simulink model "PlantVDBS1"  (R2023a)
settings: Solver=VariableStepAuto  StartTime=0.0  StopTime=10  MaxStep=0.002  RelTol=1e-6
undefined symbols (not defined in the file): c, C, C_alpha_f, C_col, C_r, E, e_c, F_zf, F_zr, J_col, K, l_f, l_r, m, n_st, t_0, T_f
libraries: autolibshared x1
settings Model: Creator=Tan_Tram  LastModifiedBy=Tan_Tram

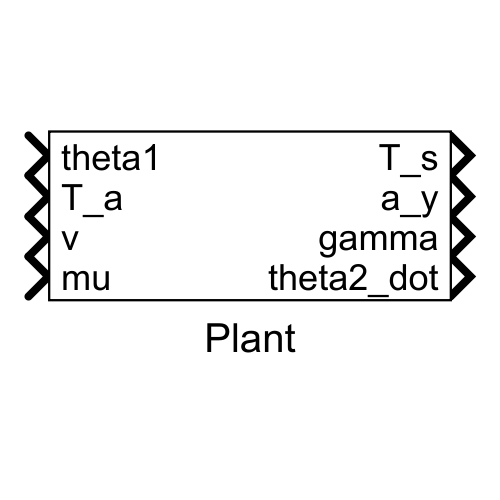
[thumbnail: Simulink's stored preview of the top-level diagram]
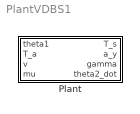
== system PlantVDBS1 ==
  Plant : Subsystem

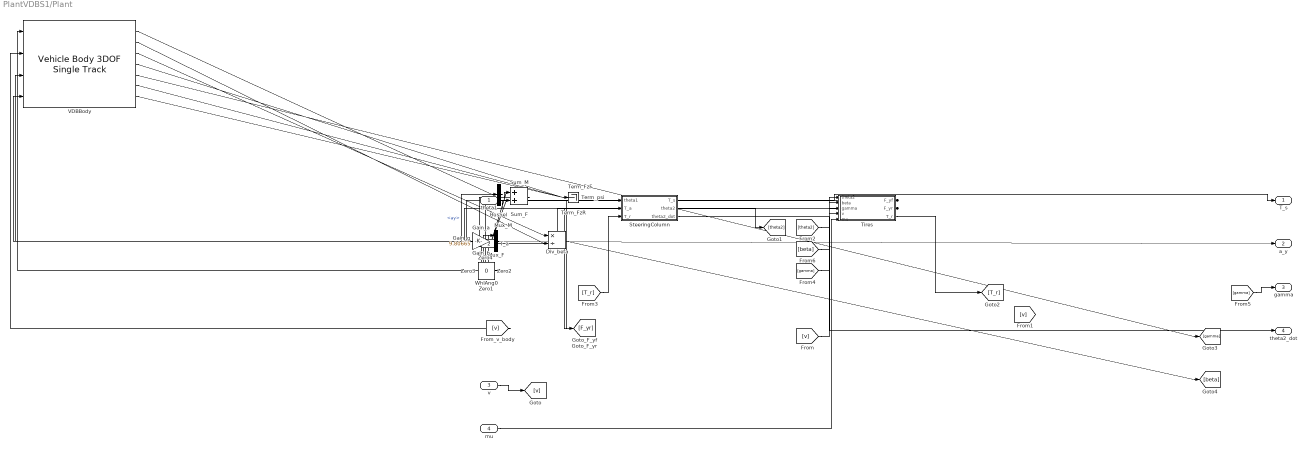
== system PlantVDBS1/Plant ==
  theta1 : Inport
  T_a : Inport  Port=2
  v : Inport  Port=3
  mu : Inport  Port=4
  BusSel : BusSelector  OutputSignals=BdyFrm.Cg.Acc.ay
  Div_beta : Product  Inputs=*/
  Gain_a : Gain  Gain=l_f
  Gain_b : Gain  Gain=l_r
  Gain_g : Gain  Gain=9.80665
  Mux_F : Mux  Inputs=3
  Mux_M : Mux  Inputs=3
  SteeringColumn : Subsystem
  Sum_F : Sum
  Sum_M : Sum  Inputs=+-
  Term_FzF : Terminator
  Term_FzR : Terminator
  Term_psi : Terminator
  Tires : Subsystem
  VDBBody : autolibshared/Vehicle Body 3DOF Single Track  trackMode=Single (bicycle)  inputMode=External longitudinal velocity  frontSteerMode=on  rearSteerMode=off  windMode=off  muMode=off  extFMode=on  extMMode=on  htchFMode=off  htchMMode=off  extXo=off  extpsio=off  extxdoto=off  extro=off  extYo=off  extTamb=off  extydoto=off  aMode=2  NF=2  NR=2  m=m  a=l_f  b=l_r  h=0.35  dh=1  hh=0.2  X_o=0  xdot_o=vdb_v0  CalphaMode=off  sigmaMode=off  d=0  hl=0  w=[1.4,1.4]  Cy_f=0  Cy_r=0  sigma_f=.1  sigma_r=.1  alpha_f_brk=[-.1 .1]  Cy_f_data=[-9e3 9e3]  alpha_r_brk=[-.1 .1]  Cy_r_data=[-9e3 9e3]  Y_o=0  ydot_o=0  Izz=Iz  psi_o=0  r_o=0  Af=2  Cd=0  Cl=0  Cpm=0  beta_w=[0 0.01:0.01:0.3]  Cs=[0 0 0 0 0 0 0 0 0 0 0 0 0 0 0 0 0 0 0 0 0 0 0 0 0 0 0 0 0 0 0]  Cym=[0 0 0 0 0 0 0 0 0 0 0 0 0 0 0 0 0 0 0 0 0 0 0 0 0 0 0 0 0 0 0]  Pabs=101325  Tair=273  g=9.81  mu=1  xdot_tol=.01  Fznom=5000  Fxtire_sat=7e4  Fytire_sat=7e4  longOff=0  latOff=0  vertOff=0  wrapAng=off
  WhlAng0 : Constant  Value=0
  Zero{1..4} (4 alike) : Constant  Value=0
  T_s : Outport
  a_y : Outport  Port=2
  gamma : Outport  Port=3
  theta2_dot : Outport  Port=4
  wires:
  [beta] -> Tires/2(beta)
  [gamma] -> gamma/1
  [gamma] -> Tires/3(gamma)
  [T_r] -> SteeringColumn/3(T_r)
  Tires/3(T_r) -> [T_r]
  [theta2] -> Tires/1(theta2)
  SteeringColumn/2(theta2) -> [theta2]
  [v] -> Tires/4(v)
  v/1 -> [v]
  SteeringColumn/3(theta2_dot) -> theta2_dot/1
  SteeringColumn/1(T_s) -> T_s/1
  mu/1 -> Tires/5(mu)
  T_a/1 -> SteeringColumn/2(T_a)
  theta1/1 -> SteeringColumn/1(theta1)
  Tires/1(F_yf) -> [F_yf], Sum_F/1, Gain_a/1
  Tires/2(F_yr) -> [F_yr], Sum_F/2, Gain_b/1
  Zero1/1 -> Mux_F/1
  Sum_F/1 -> Mux_F/2
  Zero2/1 -> Mux_F/3
  Gain_a/1 -> Sum_M/1
  Gain_b/1 -> Sum_M/2
  Zero3/1 -> Mux_M/1
  Zero4/1 -> Mux_M/2
  Sum_M/1 -> Mux_M/3
  WhlAng0/1 -> VDBBody/1
  Mux_F/1 -> VDBBody/3
  Mux_M/1 -> VDBBody/4
  [v] -> VDBBody/2
  VDBBody/3 -> Div_beta/1
  VDBBody/2 -> Div_beta/2
  Div_beta/1 -> [beta]
  VDBBody/5 -> [gamma]
  VDBBody/1 -> BusSel/1
  BusSel/1 -> Gain_g/1  "<ay>"
  Gain_g/1 -> a_y/1
  VDBBody/4 -> Term_psi/1
  VDBBody/6 -> Term_FzF/1
  VDBBody/7 -> Term_FzR/1

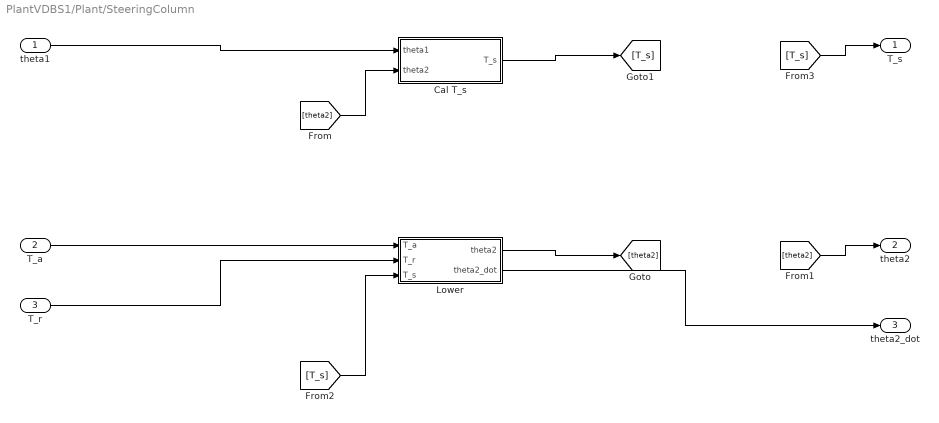
== system PlantVDBS1/Plant/SteeringColumn ==
  theta1 : Inport
  T_a : Inport  Port=2
  T_r : Inport  Port=3
  Cal T_s : Subsystem
  Lower : Subsystem
  T_s : Outport
  theta2 : Outport  Port=2
  theta2_dot : Outport  Port=3
  wires:
  theta1/1 -> Cal T_s/1(theta1)
  T_a/1 -> Lower/1(T_a)
  T_r/1 -> Lower/2(T_r)
  Lower/2(theta2_dot) -> theta2_dot/1
  Lower/1(theta2) -> [theta2]
  [theta2] -> Cal T_s/2(theta2)
  [theta2] -> theta2/1
  Cal T_s/1(T_s) -> [T_s]
  [T_s] -> Lower/3(T_s)
  [T_s] -> T_s/1

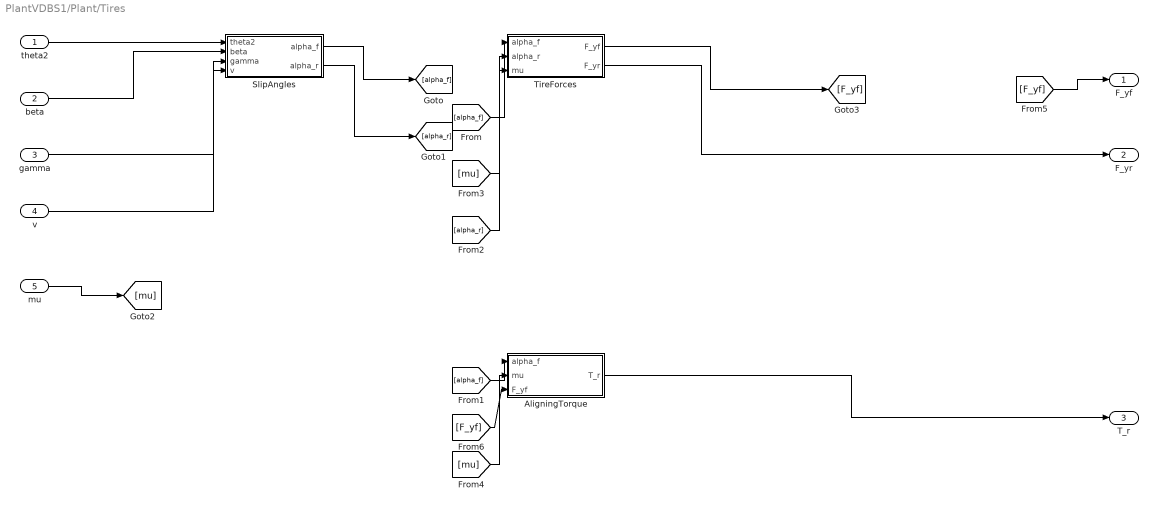
== system PlantVDBS1/Plant/Tires ==
  theta2 : Inport
  beta : Inport  Port=2
  gamma : Inport  Port=3
  v : Inport  Port=4
  mu : Inport  Port=5
  AligningTorque : Subsystem
  SlipAngles : Subsystem
  TireForces : Subsystem
  F_yf : Outport
  F_yr : Outport  Port=2
  T_r : Outport  Port=3
  wires:
  theta2/1 -> SlipAngles/1(theta2)
  beta/1 -> SlipAngles/2(beta)
  gamma/1 -> SlipAngles/3(gamma)
  v/1 -> SlipAngles/4(v)
  SlipAngles/1(alpha_f) -> [alpha_f]
  [alpha_f] -> TireForces/1(alpha_f)
  [alpha_f] -> AligningTorque/1(alpha_f)
  SlipAngles/2(alpha_r) -> [alpha_r]
  [alpha_r] -> TireForces/2(alpha_r)
  mu/1 -> [mu]
  [mu] -> TireForces/3(mu)
  [mu] -> AligningTorque/2(mu)
  TireForces/1(F_yf) -> [F_yf]
  [F_yf] -> F_yf/1
  [F_yf] -> AligningTorque/3(F_yf)
  TireForces/2(F_yr) -> F_yr/1
  AligningTorque/1(T_r) -> T_r/1

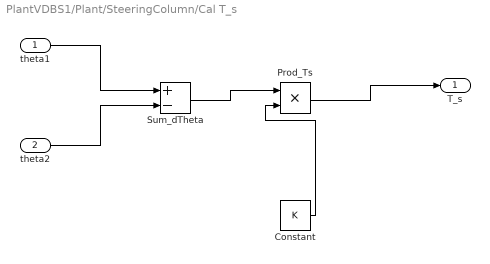
== system PlantVDBS1/Plant/SteeringColumn/Cal T_s ==
  theta1 : Inport
  theta2 : Inport  Port=2
  Constant : Constant  Value=K
  Prod_Ts : Product  Inputs=**
  Sum_dTheta : Sum  Inputs=+-
  T_s : Outport
  wires:
  theta1/1 -> Sum_dTheta/1
  theta2/1 -> Sum_dTheta/2
  Sum_dTheta/1 -> Prod_Ts/1
  Constant/1 -> Prod_Ts/2
  Prod_Ts/1 -> T_s/1

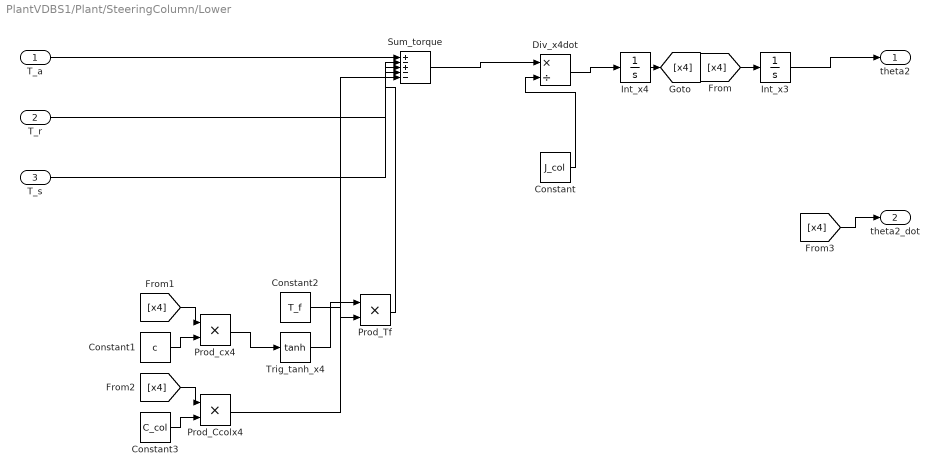
== system PlantVDBS1/Plant/SteeringColumn/Lower ==
  T_a : Inport
  T_r : Inport  Port=2
  T_s : Inport  Port=3
  Constant : Constant  Value=J_col
  Constant1 : Constant  Value=c
  Constant2 : Constant  Value=T_f
  Constant3 : Constant  Value=C_col
  Div_x4dot : Product  Inputs=*/
  Int_x3 : Integrator
  Int_x4 : Integrator
  Prod_Ccolx4 : Product  Inputs=**
  Prod_Tf : Product  Inputs=**
  Prod_cx4 : Product  Inputs=**
  Sum_torque : Sum  Inputs=+-+--
  Trig_tanh_x4 : Trigonometry  Operator=tanh
  theta2 : Outport
  theta2_dot : Outport  Port=2
  wires:
  Int_x4/1 -> [x4]
  [x4] -> Prod_cx4/1
  Constant1/1 -> Prod_cx4/2
  Prod_cx4/1 -> Trig_tanh_x4/1
  Trig_tanh_x4/1 -> Prod_Tf/1
  Constant2/1 -> Prod_Tf/2
  [x4] -> Prod_Ccolx4/1
  Constant3/1 -> Prod_Ccolx4/2
  T_a/1 -> Sum_torque/1
  T_r/1 -> Sum_torque/2
  T_s/1 -> Sum_torque/3
  Prod_Tf/1 -> Sum_torque/4
  Prod_Ccolx4/1 -> Sum_torque/5
  Sum_torque/1 -> Div_x4dot/1
  Constant/1 -> Div_x4dot/2
  Div_x4dot/1 -> Int_x4/1
  [x4] -> Int_x3/1
  Int_x3/1 -> theta2/1
  [x4] -> theta2_dot/1

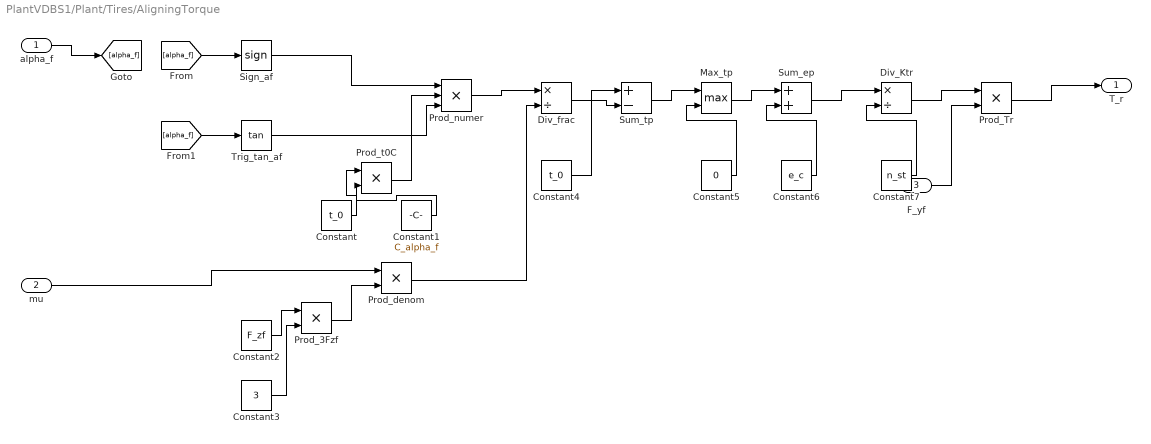
== system PlantVDBS1/Plant/Tires/AligningTorque ==
  alpha_f : Inport
  mu : Inport  Port=2
  F_yf : Inport  Port=3
  Constant : Constant  Value=t_0
  Constant1 : Constant  Value=C_alpha_f
  Constant2 : Constant  Value=F_zf
  Constant3 : Constant  Value=3
  Constant4 : Constant  Value=t_0
  Constant5 : Constant  Value=0
  Constant6 : Constant  Value=e_c
  Constant7 : Constant  Value=n_st
  Div_Ktr : Product  Inputs=*/
  Div_frac : Product  Inputs=*/
  Max_tp : MinMax  Function=max  Inputs=2
  Prod_3Fzf : Product  Inputs=**
  Prod_Tr : Product  Inputs=**
  Prod_denom : Product  Inputs=**
  Prod_numer : Product  Inputs=***
  Prod_t0C : Product  Inputs=**
  Sign_af : Signum
  Sum_ep : Sum
  Sum_tp : Sum  Inputs=+-
  Trig_tan_af : Trigonometry  Operator=tan
  T_r : Outport
  wires:
  alpha_f/1 -> [alpha_f]
  [alpha_f] -> Sign_af/1
  [alpha_f] -> Trig_tan_af/1
  Constant/1 -> Prod_t0C/1
  Constant1/1 -> Prod_t0C/2
  Sign_af/1 -> Prod_numer/1
  Prod_t0C/1 -> Prod_numer/2
  Trig_tan_af/1 -> Prod_numer/3
  Constant2/1 -> Prod_3Fzf/1
  Constant3/1 -> Prod_3Fzf/2
  mu/1 -> Prod_denom/1
  Prod_3Fzf/1 -> Prod_denom/2
  Prod_numer/1 -> Div_frac/1
  Prod_denom/1 -> Div_frac/2
  Constant4/1 -> Sum_tp/1
  Div_frac/1 -> Sum_tp/2
  Sum_tp/1 -> Max_tp/1
  Constant5/1 -> Max_tp/2
  Max_tp/1 -> Sum_ep/1
  Constant6/1 -> Sum_ep/2
  Sum_ep/1 -> Div_Ktr/1
  Constant7/1 -> Div_Ktr/2
  Div_Ktr/1 -> Prod_Tr/1
  F_yf/1 -> Prod_Tr/2
  Prod_Tr/1 -> T_r/1

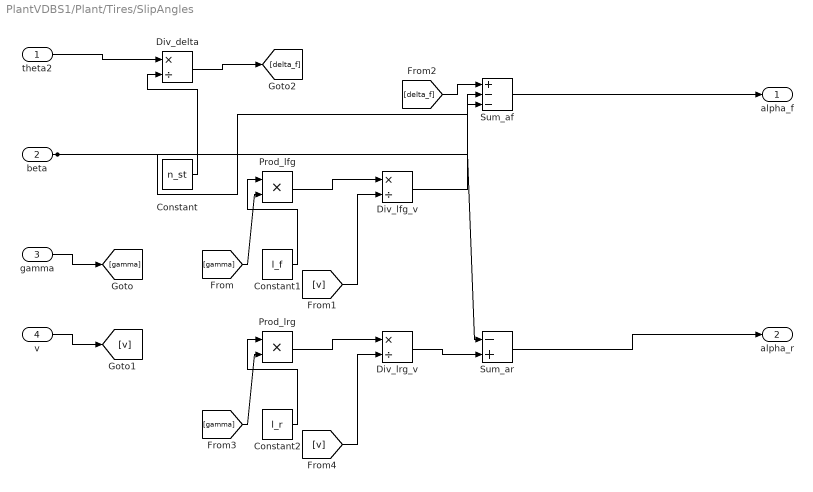
== system PlantVDBS1/Plant/Tires/SlipAngles ==
  theta2 : Inport
  beta : Inport  Port=2
  gamma : Inport  Port=3
  v : Inport  Port=4
  Constant : Constant  Value=n_st
  Constant1 : Constant  Value=l_f
  Constant2 : Constant  Value=l_r
  Div_delta : Product  Inputs=*/
  Div_lfg_v : Product  Inputs=*/
  Div_lrg_v : Product  Inputs=*/
  Prod_lfg : Product  Inputs=**
  Prod_lrg : Product  Inputs=**
  Sum_af : Sum  Inputs=+--
  Sum_ar : Sum  Inputs=-+
  alpha_f : Outport
  alpha_r : Outport  Port=2
  wires:
  gamma/1 -> [gamma]
  v/1 -> [v]
  theta2/1 -> Div_delta/1
  Constant/1 -> Div_delta/2
  Constant1/1 -> Prod_lfg/1
  [gamma] -> Prod_lfg/2
  Prod_lfg/1 -> Div_lfg_v/1
  [v] -> Div_lfg_v/2
  Div_delta/1 -> [delta_f]
  [delta_f] -> Sum_af/1
  beta/1 -> Sum_af/2, Sum_ar/1
  Div_lfg_v/1 -> Sum_af/3
  Sum_af/1 -> alpha_f/1
  Constant2/1 -> Prod_lrg/1
  [gamma] -> Prod_lrg/2
  Prod_lrg/1 -> Div_lrg_v/1
  [v] -> Div_lrg_v/2
  Div_lrg_v/1 -> Sum_ar/2
  Sum_ar/1 -> alpha_r/1

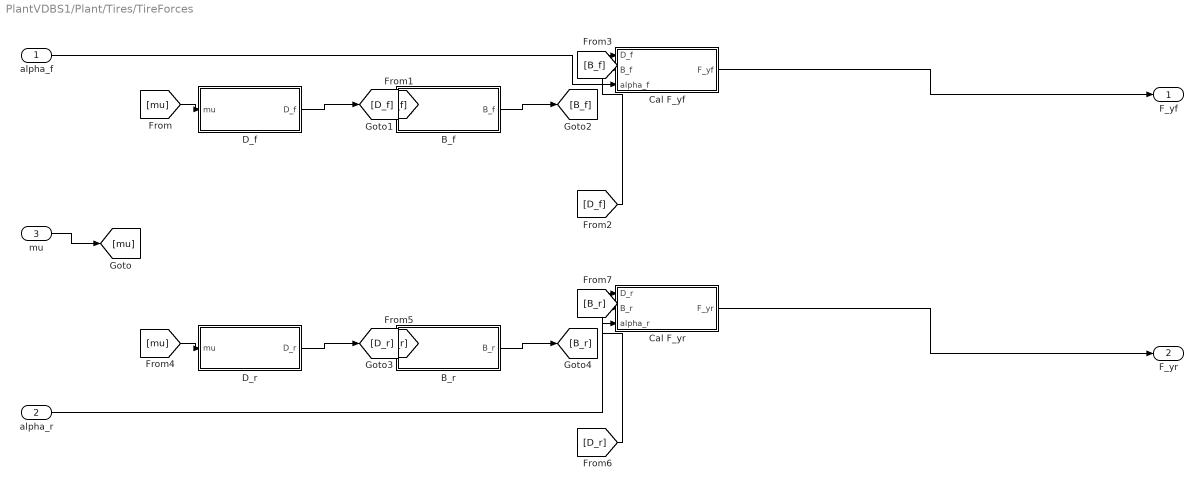
== system PlantVDBS1/Plant/Tires/TireForces ==
  alpha_f : Inport
  alpha_r : Inport  Port=2
  mu : Inport  Port=3
  B_f : Subsystem
  B_r : Subsystem
  Cal F_yf : Subsystem
  Cal F_yr : Subsystem
  D_f : Subsystem
  D_r : Subsystem
  F_yf : Outport
  F_yr : Outport  Port=2
  wires:
  mu/1 -> [mu]
  [mu] -> D_f/1(mu)
  D_f/1(D_f) -> [D_f]
  [D_f] -> B_f/1(D_f)
  [D_f] -> Cal F_yf/1(D_f)
  B_f/1(B_f) -> [B_f]
  [B_f] -> Cal F_yf/2(B_f)
  alpha_f/1 -> Cal F_yf/3(alpha_f)
  Cal F_yf/1(F_yf) -> F_yf/1
  [mu] -> D_r/1(mu)
  D_r/1(D_r) -> [D_r]
  [D_r] -> B_r/1(D_r)
  [D_r] -> Cal F_yr/1(D_r)
  B_r/1(B_r) -> [B_r]
  [B_r] -> Cal F_yr/2(B_r)
  alpha_r/1 -> Cal F_yr/3(alpha_r)
  Cal F_yr/1(F_yr) -> F_yr/1

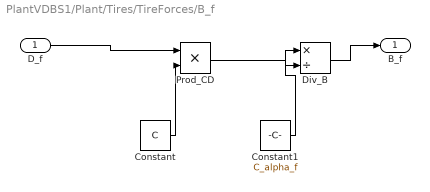
== system PlantVDBS1/Plant/Tires/TireForces/B_f ==
  D_f : Inport
  Constant : Constant  Value=C
  Constant1 : Constant  Value=C_alpha_f
  Div_B : Product  Inputs=*/
  Prod_CD : Product  Inputs=**
  B_f : Outport
  wires:
  D_f/1 -> Prod_CD/1
  Constant/1 -> Prod_CD/2
  Constant1/1 -> Div_B/1
  Prod_CD/1 -> Div_B/2
  Div_B/1 -> B_f/1

== system PlantVDBS1/Plant/Tires/TireForces/B_r ==
  D_r : Inport
  Constant : Constant  Value=C
  Constant1 : Constant  Value=C_r
  Div_B : Product  Inputs=*/
  Prod_CD : Product  Inputs=**
  B_r : Outport
  wires:
  D_r/1 -> Prod_CD/1
  Constant/1 -> Prod_CD/2
  Constant1/1 -> Div_B/1
  Prod_CD/1 -> Div_B/2
  Div_B/1 -> B_r/1

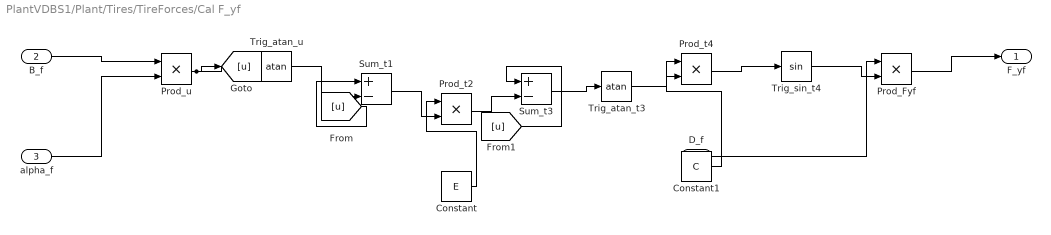
== system PlantVDBS1/Plant/Tires/TireForces/Cal F_yf ==
  D_f : Inport
  B_f : Inport  Port=2
  alpha_f : Inport  Port=3
  Constant : Constant  Value=E
  Constant1 : Constant  Value=C
  Prod_Fyf : Product  Inputs=**
  Prod_t2 : Product  Inputs=**
  Prod_t4 : Product  Inputs=**
  Prod_u : Product  Inputs=**
  Sum_t1 : Sum  Inputs=+-
  Sum_t3 : Sum  Inputs=+-
  Trig_atan_t3 : Trigonometry  Operator=atan
  Trig_atan_u : Trigonometry  Operator=atan
  Trig_sin_t4 : Trigonometry
  F_yf : Outport
  wires:
  B_f/1 -> Prod_u/1
  alpha_f/1 -> Prod_u/2
  Prod_u/1 -> Trig_atan_u/1, [u]
  [u] -> Sum_t1/1
  Trig_atan_u/1 -> Sum_t1/2
  Constant/1 -> Prod_t2/1
  Sum_t1/1 -> Prod_t2/2
  [u] -> Sum_t3/1
  Prod_t2/1 -> Sum_t3/2
  Sum_t3/1 -> Trig_atan_t3/1
  Constant1/1 -> Prod_t4/1
  Trig_atan_t3/1 -> Prod_t4/2
  Prod_t4/1 -> Trig_sin_t4/1
  D_f/1 -> Prod_Fyf/1
  Trig_sin_t4/1 -> Prod_Fyf/2
  Prod_Fyf/1 -> F_yf/1

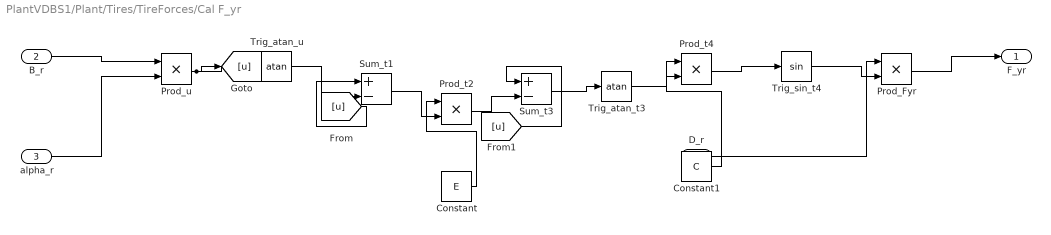
== system PlantVDBS1/Plant/Tires/TireForces/Cal F_yr ==
  D_r : Inport
  B_r : Inport  Port=2
  alpha_r : Inport  Port=3
  Constant : Constant  Value=E
  Constant1 : Constant  Value=C
  Prod_Fyr : Product  Inputs=**
  Prod_t2 : Product  Inputs=**
  Prod_t4 : Product  Inputs=**
  Prod_u : Product  Inputs=**
  Sum_t1 : Sum  Inputs=+-
  Sum_t3 : Sum  Inputs=+-
  Trig_atan_t3 : Trigonometry  Operator=atan
  Trig_atan_u : Trigonometry  Operator=atan
  Trig_sin_t4 : Trigonometry
  F_yr : Outport
  wires:
  B_r/1 -> Prod_u/1
  alpha_r/1 -> Prod_u/2
  Prod_u/1 -> Trig_atan_u/1, [u]
  [u] -> Sum_t1/1
  Trig_atan_u/1 -> Sum_t1/2
  Constant/1 -> Prod_t2/1
  Sum_t1/1 -> Prod_t2/2
  [u] -> Sum_t3/1
  Prod_t2/1 -> Sum_t3/2
  Sum_t3/1 -> Trig_atan_t3/1
  Constant1/1 -> Prod_t4/1
  Trig_atan_t3/1 -> Prod_t4/2
  Prod_t4/1 -> Trig_sin_t4/1
  D_r/1 -> Prod_Fyr/1
  Trig_sin_t4/1 -> Prod_Fyr/2
  Prod_Fyr/1 -> F_yr/1

== system PlantVDBS1/Plant/Tires/TireForces/D_f ==
  mu : Inport
  Constant : Constant  Value=F_zf
  Prod_D : Product  Inputs=**
  D_f : Outport
  wires:
  mu/1 -> Prod_D/1
  Constant/1 -> Prod_D/2
  Prod_D/1 -> D_f/1

== system PlantVDBS1/Plant/Tires/TireForces/D_r ==
  mu : Inport
  Constant : Constant  Value=F_zr
  Prod_D : Product  Inputs=**
  D_r : Outport
  wires:
  mu/1 -> Prod_D/1
  Constant/1 -> Prod_D/2
  Prod_D/1 -> D_r/1
